simulink model "dcdc_buffer"  (R2026a)
settings: Solver=ode23tb  StopTime=simlength  FixedStep=tc  MaxStep=glb_time.tc
values from neighbouring files (symbols this model uses):
  afe_ctrl = ctrl_afe_setup(glb_time.ts_afe, grid_emu.omega_grid_nom)    [init_model_legacy.m]
  frequency_set = 300    [init_model_legacy.m]
  glb_time = timing_setup(fpwm_afe, trgo_afe, fpwm_inv, trgo_inv, fpwm_single_phase_inv, trgo_single_phase_inv, fpwm_dab, trgo_dab,      fpwm_psfbc, trgo_psfbc, fpwm_isop_rail, trgo_isop_rail, fpwm_cllc, trgo_cllc, t_measure, tc_factor, tc_decimation, delay_pwm, dead_time_afe,      dead_time_inv, dead_time_single_phase_inv, dead_time_dab, dead_time_psfbc, dead_time_isop_rail, dead_time_cllc)    [init_model_legacy.m]
  grid_emu = grid_three_phase_emulator('Dyn11', delta_star, grid_nominal_power, application_voltage, us1, us2, fgrid,                  eq_grid_inductance, eq_grid_resistance, eta, ucc, i1m, p_iron, n1, n2, core_area, core_length, mur,                  up_xi_pu_ref, up_eta_pu_ref, un_xi_pu_ref, un_eta_pu_ref)    [init_model_legacy.m]
  heatsink = liquid_cooled_plate_2kw_setup(weight, no_weight, cp_al, heat_capacity_hs, thermal_conductivity_al,      Rth_switch_HA, Rth_mosfet_HA, Rth_diode_HA, Tambient, DThs_init)    [init_model_legacy.m]
  Tambient = 40    [init_model_legacy.m]
undefined symbols (not defined in the file or in its folder): hwdata, igbt, magnitude
libraries: fl_lib x113, nesl_utility x63, igbt_simple_2th_lib x4, ee_lib x2, pi_ctrl x2, dq_vector_pi x1, linear_double_integrator_observer_ccaller x1, phase_shift_filter_ccaller x1, discrete_time_low_pass_filter x1, single_phase_pwm_modulator x1, three_phase_voltage_with_frt_emulator x1
(part 1 of 4)
settings Model: SimulationMode=accelerator  Creator=LTNBDA  LastModifiedBy=ltnbda
settings SolverCC: ZeroCrossControl=DisableAll  ZeroCrossAlgorithm=Adaptive  SolverResetMethod=Robust
settings DataIOCC: MaxDataPoints=1  SignalLoggingSaveFormat=ModelDataLogs
settings OptimizationCC: InitFltsAndDblsToZero=on  EfficientMapNaN2IntZero=off
settings DebuggingCC: SaveWithParameterizedLinksMsg=none  SignalResolutionControl=TryResolveAllWithWarning  IgnoredZcDiagnostic=none  MultiTaskDSMMsg=warning  MultiTaskCondExecSysMsg=none  MultiTaskRateTransMsg=warning
settings HardwareCC: ProdBitPerLong=64.0  ProdHWDeviceType=Generic->64-bit Embedded Processor (LP64)  TargetBitPerPointer=64.0  TargetBitPerSizeT=64.0  TargetBitPerPtrDiffT=64.0  TargetLongLongMode=on  TargetIntDivRoundTo=Zero  TargetEndianess=LittleEndian  TargetWordSize=64.0  TargetHWDeviceType=MATLAB Host  ProdEqTarget=off
settings SFSimCC: SimCustomHeaderCode=|
  | #include "phase_shift_flt_simulink.h"
  | #include "sv_pwm.h"
  | #include "rpi.h"
  | #include "rpi_simulink.h"
  | #include "first_harmonic_tracker.h"
  | #include "dqvector_pi.h"
  | #include "dqvector_pi_simulink.h"
  | #include "sv_pwm_simulink.h"
  | #include "dqpll_grid.h"
  | #include "first_harmonic_tracker_simulink.h"
  | #include "dqpll_grid_simulink.h"
  | #include "phase_shift_flt.h"
  | #include "math_f.h"
  | #include "linear_double_integrator_observer_simulink.h"
  | #include "linear_double_integrator_observer.h"
  | #include "sogi_flt_simulink.h"
  | #include "sogi_flt.h"
settings SFSimCC: SimUserSources=|
  | "rpi.c"
  | "rpi_simulink.c"
  | "dqvector_pi_simulink.c"
  | "dqvector_pi.c"
  | "sv_pwm_simulink.c"
  | "sv_pwm.c"
  | "first_harmonic_tracker_simulink.c"
  | "first_harmonic_tracker.c"
  | "dqpll_grid_simulink.c"
  | "dqpll_grid.c"
  | "phase_shift_flt_simulink.c"
  | "phase_shift_flt.c"
  | "linear_double_integrator_observer_simulink.c"
  | "linear_double_integrator_observer.c"
  | "sogi_flt_simulink.c"
  | "sogi_flt.c"
settings SFSimCC: SimUserIncludeDirs=|
  | include
  | src
settings CodeAppCC: MaxIdLength=128.0
settings GRTTargetCC: CombineOutputUpdateFcns=off  GRTInterface=on
settings SimscapeCC: SimscapeNormalizeSystem=off  SimscapeNominalValues="[{\"value\":\"1\",\"unit\":\"A\"},{\"value\":\"1\",\"unit\":\"bar\"},{\"value\":\"1\",\"unit\":\"cm^2\"},{\"value\":\"1\",\"unit\":\"cm^3/s\"},{\"value\":\"1\",\"unit\":\"kJ/kg\"},{\"value\":\"1\",\"unit\":\"kW\"},{\"value\":\"1\",\"unit\":\"l\"},{\"value\":\"1\",\"unit\":\"N\"},{\"value\":\"1\",\"unit\":\"N*m\"},{\"value\":\"1\",\"unit\":\"V\"}]"  SimscapeLogType=none  SimscapeLogDataHistory=5000.0

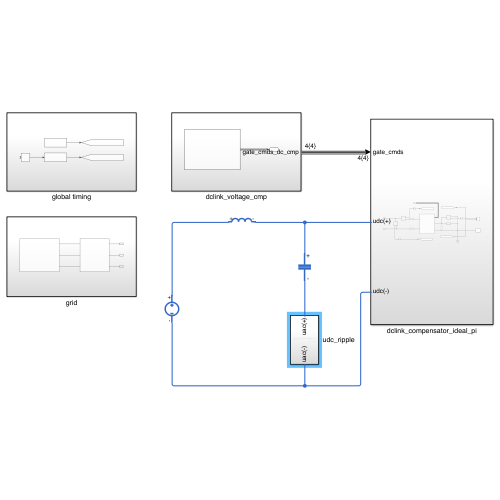
[thumbnail: Simulink's stored preview of the top-level diagram]
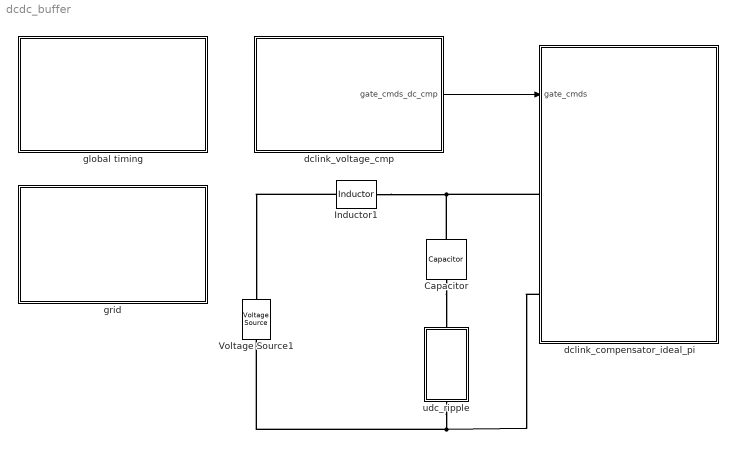
== system dcdc_buffer ==
  Capacitor : fl_lib/Electrical/Electrical Elements/Capacitor  c=7.2e-3 F  r=1e-6 Ohm  g=0 1/Ohm  i_specify=off  i_priority=None  i=0 A  i_nominal_specify=off  i_nominal_value=1  i_nominal_unit=A  v_specify=off  v_priority=None  v=0 V  v_nominal_specify=off  v_nominal_value=1  v_nominal_unit=V  vc_specify=off  vc_priority=High  vc=0 V  vc_nominal_specify=off  vc_nominal_value=1  vc_nominal_unit=V
  Inductor1 : fl_lib/Electrical/Electrical Elements/Inductor  l=250e-6 H  r=50e-3 Ohm  g=1e-9 1/Ohm  i_specify=off  i_priority=None  i=0 A  i_nominal_specify=off  i_nominal_value=1  i_nominal_unit=A  v_specify=off  v_priority=None  v=0 V  v_nominal_specify=off  v_nominal_value=1  v_nominal_unit=V  i_L_specify=off  i_L_priority=High  i_L=0 A  i_L_nominal_specify=off  i_L_nominal_value=1  i_L_nominal_unit=A
  Voltage Source1 : ee_lib/Sources/Voltage Source  dc_voltage=hwdata.single_phase_inverter.udc_nom V  ac_voltage=0 V  ac_shift=0 rad  ac_frequency=0 Hz  noise_mode=ee.enum.sources.noise.Disabled  PSD=0 V^2/Hz  sample_time=1e-3 s  repeatability=ee.enum.sources.repeatability.NotRepeatable  user_seed=0  auto_seed=3890346746  i_specify=off  i_priority=None  i=0 A  i_nominal_specify=off  i_nominal_value=1  i_nominal_unit=A  v_specify=off  v_priority=None  v=0 V  v_nominal_specify=off  v_nominal_value=1  v_nominal_unit=V
  dclink_compensator_ideal_pi : Subsystem
  dclink_voltage_cmp : Subsystem
  global timing : Subsystem
  grid : Subsystem
  udc_ripple : Subsystem
  wires:
  dclink_voltage_cmp/1(gate_cmds_dc_cmp) -> dclink_compensator_ideal_pi/1(gate_cmds)
  connections:
  dclink_compensator_ideal_pi/LConn1 -- Inductor1/RConn1 -- Capacitor/LConn1
  Inductor1/LConn1 -- Voltage Source1/LConn1
  Capacitor/RConn1 -- udc_ripple/LConn1
  udc_ripple/RConn1 -- Voltage Source1/RConn1 -- dclink_compensator_ideal_pi/LConn2

== system dcdc_buffer/dclink_compensator_ideal_pi ==
  gate_cmds : Inport
  Capacitor : fl_lib/Electrical/Electrical Elements/Capacitor  c=12e-3 F  r=1e-6 Ohm  g=0 1/Ohm  i_specify=off  i_priority=None  i=0 A  i_nominal_specify=off  i_nominal_value=1  i_nominal_unit=A  v_specify=off  v_priority=None  v=0 V  v_nominal_specify=off  v_nominal_value=1  v_nominal_unit=V  vc_specify=off  vc_priority=High  vc=0 V  vc_nominal_specify=off  vc_nominal_value=1  vc_nominal_unit=V
  Current Sensor : fl_lib/Electrical/Electrical Sensors/Current Sensor
  Electrical Reference1 : fl_lib/Electrical/Electrical Elements/Electrical Reference
  Inductor : fl_lib/Electrical/Electrical Elements/Inductor  l=250e-6 H  r=4e-3 Ohm  g=1e-9 1/Ohm  i_specify=off  i_priority=None  i=0 A  i_nominal_specify=off  i_nominal_value=1  i_nominal_unit=A  v_specify=off  v_priority=None  v=0 V  v_nominal_specify=off  v_nominal_value=1  v_nominal_unit=V  i_L_specify=off  i_L_priority=High  i_L=0 A  i_L_nominal_specify=off  i_L_nominal_value=1  i_L_nominal_unit=A
  Inductor1 : fl_lib/Electrical/Electrical Elements/Inductor  l=250e-6 H  r=4e-3 Ohm  g=1e-9 1/Ohm  i_specify=off  i_priority=None  i=0 A  i_nominal_specify=off  i_nominal_value=1  i_nominal_unit=A  v_specify=off  v_priority=None  v=0 V  v_nominal_specify=off  v_nominal_value=1  v_nominal_unit=V  i_L_specify=off  i_L_priority=High  i_L=0 A  i_L_nominal_specify=off  i_L_nominal_value=1  i_L_nominal_unit=A
  PS-Simulink Converter : nesl_utility/PS-Simulink Converter  PhysicalDomain=network_engine_domain  SubClassName=ps_output  LeftPortType=input  RightPortType=output  PseudoPeriodic=off  Frequencies=[]  VectorFormat=1-D array  Unit=A  AffineConversion=off
  PS-Simulink Converter1 : nesl_utility/PS-Simulink Converter  PhysicalDomain=network_engine_domain  SubClassName=ps_output  LeftPortType=input  RightPortType=output  PseudoPeriodic=off  Frequencies=[]  VectorFormat=1-D array  Unit=V  AffineConversion=off
  PS-Simulink Converter2 : nesl_utility/PS-Simulink Converter  PhysicalDomain=network_engine_domain  SubClassName=ps_output  LeftPortType=input  RightPortType=output  PseudoPeriodic=off  Frequencies=[]  VectorFormat=1-D array  Unit=V  AffineConversion=off
  Solver Configuration : nesl_utility/Solver Configuration  PhysicalDomain=network_engine_domain  SubClassName=solver  LeftPortType=input  RightPortType=generic  Tones=[]  Harmonics=[]  SimulateNoise=off  Profile=off  UseLocalSampling=off  EnableSwitchedLinearOptims=on  FrequencyDomain=off  UseCCode=off  RelTol=0.001  AbsTol=0.001  MinStep=1e-09  ToWorkspace=off  RevertToSquareIcSolve=off  NumHomotopyIterations=100  PhasorMode=off  PhasorModeNumHarmonics=1  ConsistencySolver=NEWTON_FTOL  CanonicalOrdering=UNORDERED  OptimizeIntermediates=UNOPTIMIZED  IndexReductionMethod=DerivativeReplacement  DoDC=off  ResidualTolerance=1e-4  ConsistencyTolSource=GLOBAL  ConsistencyAbsTol=0.001  ConsistencyRelTol=0.001  ConsistencyTolFactor=0.001  UseLocalSolver=on  LocalSolverChoice=NE_BACKWARD_EULER_ADVANCER  ResolveIndetEquations=on  FunctionEvalNumThread=1  LocalSolverSampleTime=glb_time.tc  DoFixedCost=on  MaxNonlinIter=nonlinear_iterations  MaxModeIter=2  ComputeImpulses=off  ImpulseIterations=2  LinearAlgebra=auto  LinearAlgebraNumThread=0  EquationFormulation=NE_TIME_EF  DelaysMemoryBudget=1024  AutomaticFiltering=on  FilteringTimeConstant=0.001  PartitionStorageMethod=AS_NEEDED  PartitionMemoryBudget=1024  PartitionMethod=ROBUST  MultibodyUseLocalSolver=off  MultibodyLocalSolverChoice=ODE1  MultibodyLocalSolverSampleTime=0.001
  Voltage Sensor : fl_lib/Electrical/Electrical Sensors/Voltage Sensor
  Voltage Sensor1 : fl_lib/Electrical/Electrical Sensors/Voltage Sensor
  Voltage Source : ee_lib/Sources/Voltage Source  Commented=on  dc_voltage=2000 V  ac_voltage=0 V  ac_shift=0 rad  ac_frequency=0 Hz  noise_mode=ee.enum.sources.noise.Disabled  PSD=0 V^2/Hz  sample_time=1e-3 s  repeatability=ee.enum.sources.repeatability.NotRepeatable  user_seed=0  auto_seed=3499211588  i_specify=off  i_priority=None  i=0 A  i_nominal_specify=off  i_nominal_value=1  i_nominal_unit=A  v_specify=off  v_priority=None  v=0 V  v_nominal_specify=off  v_nominal_value=1  v_nominal_unit=V
  single_phase_inverter : Subsystem
  udc_buffer : Scope  NumInputPorts=2
      settings: ActiveDisplayYMinimum=-428.225155436671  ActiveDisplayYMaximum=3854.02639893004  DataLoggingVariableName=ScopeData16
  udc(+) : PMIOPort  Side=Left
  udc(-) : PMIOPort  Port=2  Side=Left
  tag scope: dclink_voltage=global, i_buffer_glb=global, udc_buffer_glb=global
  wires:
  gate_cmds/1 -> single_phase_inverter/1(gate_cmds)
  PS-Simulink Converter/1 -> [i_buffer_glb]
  PS-Simulink Converter1/1 -> [udc_buffer_glb], udc_buffer/1  "udc_buffer_glb"
  [i_buffer_glb] -> udc_buffer/2  "i_buffer_glb"
  PS-Simulink Converter2/1 -> [dclink_voltage]  "dclink_voltage"
  connections:
  Inductor1/RConn1 -- Voltage Sensor1/RConn2 -- udc(-)/RConn1
  single_phase_inverter/RConn1 -- Inductor/RConn1
  single_phase_inverter/RConn2 -- Inductor1/LConn1
  Voltage Source/LConn1 -- Voltage Sensor/LConn1 -- Capacitor/LConn1 -- single_phase_inverter/LConn1
  Voltage Source/RConn1 -- Capacitor/RConn1 -- Voltage Sensor/RConn2 -- Electrical Reference1/LConn1 -- Solver Configuration/RConn1 -- single_phase_inverter/LConn2
  Current Sensor/RConn2 -- Inductor/LConn1
  udc(+)/RConn1 -- Voltage Sensor1/LConn1 -- Current Sensor/LConn1
  Current Sensor/RConn1 -- PS-Simulink Converter/LConn1
  PS-Simulink Converter1/LConn1 -- Voltage Sensor/RConn1
  PS-Simulink Converter2/LConn1 -- Voltage Sensor1/RConn1

== system dcdc_buffer/dclink_voltage_cmp ==
  dclink_cmp : Subsystem
  gate_cmds_dc_cmp : Outport
  wires:
  dclink_cmp/1(gate_cmds_dc_comp) -> gate_cmds_dc_cmp/1

== system dcdc_buffer/global timing ==
  Unit Delay : UnitDelay  SampleTime=glb_time.tc
  time_afe1 : Subsystem  mask{k=1}
      mask prompts: k "Time Gain"
      mask Display:
      | disp('time-gen');
      | port_label('input', 1, 'crt');
      | port_label('output', 1, 'tout');
  time_afe3 : Subsystem  mask{k=1}
      mask prompts: k "Time Gain"
      mask Display:
      | disp('time-gen');
      | port_label('output', 1, 'tout');
  tag scope: master_time=global, time_afe_module_1=global
  wires:
  time_afe1/1(Out1) -> [time_afe_module_1]
  time_afe3/1(Out1) -> [master_time]
  Unit Delay/1 -> time_afe1/1(correction_time)

== system dcdc_buffer/grid ==
  Open Circuit : fl_lib/Electrical/Electrical Elements/Open Circuit  v_specify=off  v_priority=None  v=0 V  v_nominal_specify=off  v_nominal_value=1  v_nominal_unit=V
  Open Circuit1 : fl_lib/Electrical/Electrical Elements/Open Circuit  v_specify=off  v_priority=None  v=0 V  v_nominal_specify=off  v_nominal_value=1  v_nominal_unit=V
  Open Circuit2 : fl_lib/Electrical/Electrical Elements/Open Circuit  v_specify=off  v_priority=None  v=0 V  v_nominal_specify=off  v_nominal_value=1  v_nominal_unit=V
  grid_emulator : Subsystem
  threephase_vi_measures : Subsystem
  connections:
  threephase_vi_measures/LConn3 -- grid_emulator/RConn3
  threephase_vi_measures/LConn1 -- grid_emulator/RConn1
  threephase_vi_measures/LConn2 -- grid_emulator/RConn2
  Open Circuit1/LConn1 -- threephase_vi_measures/RConn1
  Open Circuit2/LConn1 -- threephase_vi_measures/RConn2
  threephase_vi_measures/RConn3 -- Open Circuit/LConn1

== system dcdc_buffer/udc_ripple ==
  Constant : Constant  Value=-2*pi/3
  Controlled Voltage Source : fl_lib/Electrical/Electrical Sources/Controlled Voltage Source
  Gain : Gain  Gain=150
  Gain1 : Gain  Gain=2
  Simulink-PS Converter : nesl_utility/Simulink-PS Converter  PhysicalDomain=network_engine_domain  SubClassName=ps_input  LeftPortType=input  RightPortType=output  PseudoPeriodic=off  Frequencies=[]  NoiseDistribution=none  NoiseParameters=[]  Unit=V  AffineConversion=off  FilteringAndDerivatives=provide  SimscapeFilterOrder=1  InputFilterTimeConstant=0.001  UdotUserProvided=0
  Sin : Trigonometry
  Sum : Sum  Inputs=|++
  uac(+) : PMIOPort  Side=Left
  uac(-) : PMIOPort  Port=2  Side=Right
  wires:
  Sin/1 -> Gain/1
  Gain/1 -> Simulink-PS Converter/1
  [phase_grid_emulator] -> Sum/1
  Sum/1 -> Gain1/1
  Constant/1 -> Sum/2
  Gain1/1 -> Sin/1
  connections:
  Controlled Voltage Source/LConn1 -- uac(+)/RConn1
  Controlled Voltage Source/RConn2 -- uac(-)/RConn1
  Simulink-PS Converter/RConn1 -- Controlled Voltage Source/RConn1

== system dcdc_buffer/dclink_compensator_ideal_pi/single_phase_inverter ==
  gate_cmds : Inport
  single phase inverter : Subsystem
      settings: PortSchema="{\"entries\":[{\"content\":{\"sides\":[{\"content\":{\"connectorIds\":[\"LConn1\",\"LConn2\"]},\"type\":\"ConnectorPlacement.EquallySpacedRectSide\",\"uuid\":\"4fcf4fea-d38f-431b-8a91-be3ce9782faf\"},{\"content\":{\"connectorIds\":[\"RConn1\",\"RConn2\"],\"side\":\"RIGHT\"},\"type\":\"ConnectorPlacement.EquallySpacedRectSide\",\"uuid\":\"0aa56277-92e9-4e3b-84c7-43398254a4d8\"},{\"content\":{\"connectorIds\":[\"In1\"],\"side\":\"TOP\"},\"type\":\"ConnectorPlacement.EquallySpacedRectSide\",\"uuid\":\"5cd150dc-bcaf-4cd7-b2a8-3db203726730\"}]},\"type\":\"ConnectorPlacement.EquallySpacedConnector\",\"uuid\":\"bf8194c4-c327-4d40-bea4-f1e7617f80b4\"}],\"packageUris\":[\"http://schema.mathworks.com/mf0/Connector/R2020b\"],\"version\":\"1.0\"}"
  uac(+) : PMIOPort  Side=Right
  uac(-) : PMIOPort  Port=2  Side=Right
  udc(+) : PMIOPort  Port=3  Side=Left
  udc(-) : PMIOPort  Port=4  Side=Left
  wires:
  gate_cmds/1 -> single phase inverter/1(gate_cmds)
  connections:
  single phase inverter/RConn1 -- udc(+)/RConn1
  single phase inverter/LConn2 -- uac(-)/RConn1
  uac(+)/RConn1 -- single phase inverter/LConn1
  single phase inverter/RConn2 -- udc(-)/RConn1

== system dcdc_buffer/dclink_voltage_cmp/dclink_cmp ==
  acquisition_and_scaling_current_buffer : Subsystem
  acquisition_and_scaling_dc_voltage : Subsystem
  acquisition_and_scaling_dc_voltage_buffer : Subsystem
  acquisition_and_scaling_grid_voltage_ac : Subsystem
  dclink_compensation_ctrl : Subsystem
  phase_grid_hat : Scope  NumInputPorts=2
      settings: ActiveDisplayYMinimum=-4.986486486486486  ActiveDisplayYMaximum=5.4864864864864868
  pwm modulator_dclink_compensator : Subsystem
  gate_cmds_dc_comp : Outport
  wires:
  [TRGO_AFE_1] -> dclink_compensation_ctrl/Trigger
  [dclink_voltage] -> acquisition_and_scaling_dc_voltage/1(in)
  acquisition_and_scaling_dc_voltage/1(out) -> dclink_compensation_ctrl/1(dclink_voltage_pu)  "dclink_voltage_pu"
  [i_buffer_glb] -> acquisition_and_scaling_current_buffer/1(in)
  acquisition_and_scaling_current_buffer/1(out) -> dclink_compensation_ctrl/2(i_buffer_pu)
  pwm modulator_dclink_compensator/1(gate_cmds) -> gate_cmds_dc_comp/1
  dclink_compensation_ctrl/1(u_ctrl_buffer) -> pwm modulator_dclink_compensator/1(vout)
  [udc_buffer_glb] -> acquisition_and_scaling_dc_voltage_buffer/1(in)
  acquisition_and_scaling_dc_voltage_buffer/1(out) -> dclink_compensation_ctrl/3(udc_buffer_pu)
  [ug_abc] -> acquisition_and_scaling_grid_voltage_ac/1(in)
  acquisition_and_scaling_grid_voltage_ac/1(out) -> dclink_compensation_ctrl/4(ugrid_pu)  "ug_abc"
  dclink_compensation_ctrl/2(phase_grid_hat) -> phase_grid_hat/1  "phase_grid_hat"
  [phase_grid_emulator] -> phase_grid_hat/2

== system dcdc_buffer/global timing/time_afe1 ==
  correction_time : Inport
  Constant : Constant
  Gain : Gain  Gain=k
  Product : Product
  Sum : Sum  Inputs=|++
  time_1 : Clock
  Out1 : Outport
  wires:
  time_1/1 -> Gain/1
  Gain/1 -> Product/1
  Product/1 -> Out1/1
  correction_time/1 -> Sum/1
  Sum/1 -> Product/2
  Constant/1 -> Sum/2

== system dcdc_buffer/global timing/time_afe3 ==
  Gain : Gain  Gain=k
  time_1 : Clock
  Out1 : Outport
  wires:
  Gain/1 -> Out1/1
  time_1/1 -> Gain/1

== system dcdc_buffer/grid/grid_emulator ==
  Bus Selector : BusSelector  OutputSignals=ua_grid_emu,ub_grid_emu,uc_grid_emu
  Bus Selector1 : BusSelector  OutputSignals=gamma_grid_emulator,omega_grid_emulator
  Controlled Voltage Source : fl_lib/Electrical/Electrical Sources/Controlled Voltage Source
  Controlled Voltage Source1 : fl_lib/Electrical/Electrical Sources/Controlled Voltage Source
  Controlled Voltage Source2 : fl_lib/Electrical/Electrical Sources/Controlled Voltage Source
  Electrical Reference : fl_lib/Electrical/Electrical Elements/Electrical Reference
  Simulink-PS Converter : nesl_utility/Simulink-PS Converter  PhysicalDomain=network_engine_domain  SubClassName=ps_input  LeftPortType=input  RightPortType=output  PseudoPeriodic=off  Frequencies=[]  NoiseDistribution=none  NoiseParameters=[]  Unit=V  AffineConversion=on  FilteringAndDerivatives=provide  SimscapeFilterOrder=1  InputFilterTimeConstant=0.001  UdotUserProvided=0
  Simulink-PS Converter1 : nesl_utility/Simulink-PS Converter  PhysicalDomain=network_engine_domain  SubClassName=ps_input  LeftPortType=input  RightPortType=output  PseudoPeriodic=off  Frequencies=[]  NoiseDistribution=none  NoiseParameters=[]  Unit=V  AffineConversion=on  FilteringAndDerivatives=provide  SimscapeFilterOrder=1  InputFilterTimeConstant=0.001  UdotUserProvided=0
  Simulink-PS Converter2 : nesl_utility/Simulink-PS Converter  PhysicalDomain=network_engine_domain  SubClassName=ps_input  LeftPortType=input  RightPortType=output  PseudoPeriodic=off  Frequencies=[]  NoiseDistribution=none  NoiseParameters=[]  Unit=V  AffineConversion=on  FilteringAndDerivatives=provide  SimscapeFilterOrder=1  InputFilterTimeConstant=0.001  UdotUserProvided=0
  Solver Configuration : nesl_utility/Solver Configuration  PhysicalDomain=network_engine_domain  SubClassName=solver  LeftPortType=input  RightPortType=generic  Tones=[]  Harmonics=[]  SimulateNoise=off  Profile=off  UseLocalSampling=off  EnableSwitchedLinearOptims=on  FrequencyDomain=off  UseCCode=off  RelTol=0.001  AbsTol=0.001  MinStep=1e-09  ToWorkspace=off  RevertToSquareIcSolve=off  NumHomotopyIterations=100  PhasorMode=off  PhasorModeNumHarmonics=1  ConsistencySolver=NEWTON_FTOL  CanonicalOrdering=UNORDERED  OptimizeIntermediates=UNOPTIMIZED  IndexReductionMethod=DerivativeReplacement  DoDC=off  ResidualTolerance=1e-4  ConsistencyTolSource=GLOBAL  ConsistencyAbsTol=0.001  ConsistencyRelTol=0.001  ConsistencyTolFactor=0.001  UseLocalSolver=on  LocalSolverChoice=NE_BACKWARD_EULER_ADVANCER  ResolveIndetEquations=on  FunctionEvalNumThread=1  LocalSolverSampleTime=glb_time.tc  DoFixedCost=on  MaxNonlinIter=nonlinear_iterations  MaxModeIter=2  ComputeImpulses=off  ImpulseIterations=2  LinearAlgebra=auto  LinearAlgebraNumThread=0  EquationFormulation=NE_TIME_EF  DelaysMemoryBudget=1024  AutomaticFiltering=on  FilteringTimeConstant=0.001  PartitionStorageMethod=AS_NEEDED  PartitionMemoryBudget=1024  PartitionMethod=ROBUST  MultibodyUseLocalSolver=off  MultibodyLocalSolverChoice=ODE1  MultibodyLocalSolverSampleTime=0.001
  three_phase_voltage_source_with_frt_emulator : three_phase_voltage_with_frt_emulator/three_phase_voltage_source_with_frt_emulator  nominal_frequency_m=grid_emu.fgrid_nom  nominal_voltage_m=grid_emu.us_primary_nom  Vemu_ref_norm_m=grid_emu.Vemu_ref_norm  vp_xi_pu_m=grid_emu.up_xi_pu_ref  vp_eta_pu_m=grid_emu.up_eta_pu_ref  vn_xi_pu_m=grid_emu.un_xi_pu_ref  vn_eta_pu_m=grid_emu.un_eta_pu_ref  Am=filters.afe.SOF_50Hz.ss_c.A  Bm=filters.afe.SOF_50Hz.ss_c.B  Cm=filters.afe.SOF_50Hz.ss_c.C  enable_frt_1_m=frt_data.enable_frt_1  enable_frt_2_m=frt_data.enable_frt_2  start_time_LVRT_m=frt_data.start_time_LVRT  end_time_LVRT_m=frt_data.end_time_LVRT  deepPOSxi_m=frt_data.deepPOSxi  deepPOSeta_m=frt_data.deepPOSeta  deepNEGxi_m=frt_data.deepNEGxi  deepNEGeta_m=frt_data.deepNEGeta  Amplitude_U_m=frt_data.Amplitude_U  Amplitude_V_m=frt_data.Amplitude_V  Amplitude_W_m=frt_data.Amplitude_W  t_ramp_m=frt_data.t_ramp  Phase_shift_m=frt_data.Phase_shift
  threephase_vi_measures : Subsystem
  u1 : PMIOPort  Side=Right
  u2 : PMIOPort  Port=2  Side=Right
  u3 : PMIOPort  Port=3  Side=Right
  tag scope: phase_grid_emulator=global, pulsation_grid_emulator=global
  wires:
  Bus Selector1/2 -> [pulsation_grid_emulator]  "<omega_grid_emulator>"
  Bus Selector1/1 -> [phase_grid_emulator]  "<gamma_grid_emulator>"
  Bus Selector/2 -> Simulink-PS Converter1/1  "<ub_grid_emu>"
  Bus Selector/3 -> Simulink-PS Converter2/1  "<uc_grid_emu>"
  three_phase_voltage_source_with_frt_emulator/1 -> Bus Selector1/1, Bus Selector/1
  Bus Selector/1 -> Simulink-PS Converter/1  "<ua_grid_emu>"
  connections:
  Simulink-PS Converter/RConn1 -- Controlled Voltage Source/RConn1
  Simulink-PS Converter1/RConn1 -- Controlled Voltage Source1/RConn1
  Simulink-PS Converter2/RConn1 -- Controlled Voltage Source2/RConn1
  Controlled Voltage Source/RConn2 -- Controlled Voltage Source1/RConn2 -- Solver Configuration/RConn1 -- Electrical Reference/LConn1 -- Controlled Voltage Source2/RConn2
  u1/RConn1 -- threephase_vi_measures/RConn1
  u2/RConn1 -- threephase_vi_measures/RConn2
  u3/RConn1 -- threephase_vi_measures/RConn3
  Controlled Voltage Source/LConn1 -- threephase_vi_measures/LConn1
  Controlled Voltage Source1/LConn1 -- threephase_vi_measures/LConn2
  Controlled Voltage Source2/LConn1 -- threephase_vi_measures/LConn3

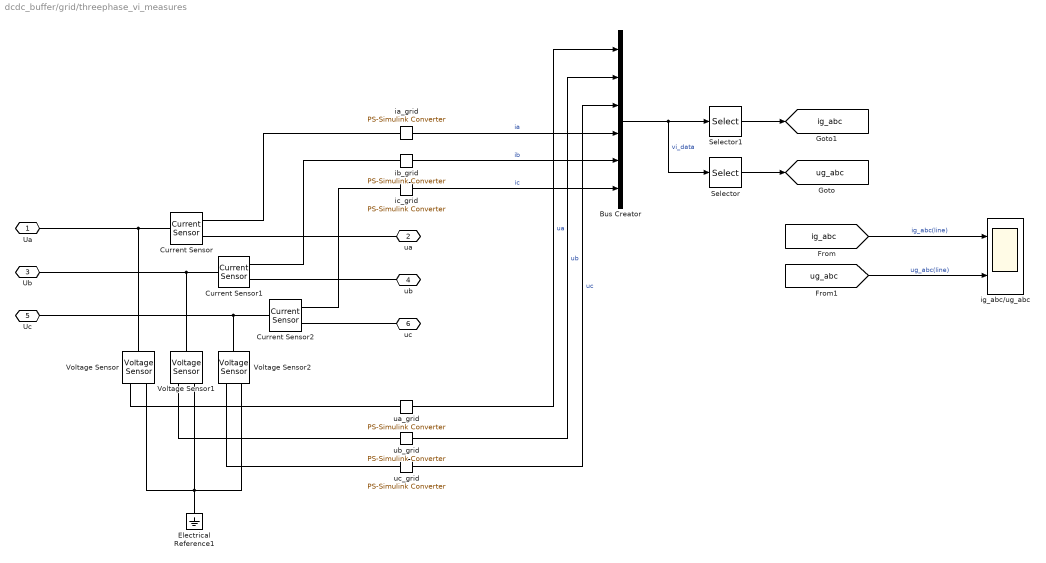
== system dcdc_buffer/grid/threephase_vi_measures ==
  Bus Creator : BusCreator  Inputs=6
  Current Sensor : fl_lib/Electrical/Electrical Sensors/Current Sensor
  Current Sensor1 : fl_lib/Electrical/Electrical Sensors/Current Sensor
  Current Sensor2 : fl_lib/Electrical/Electrical Sensors/Current Sensor
  Electrical Reference1 : fl_lib/Electrical/Electrical Elements/Electrical Reference
  Selector : Selector  InputPortWidth=6  IndexOptions=Index vector (dialog)  Indices=[1 2 3]  OutputSizes=1
  Selector1 : Selector  InputPortWidth=6  IndexOptions=Index vector (dialog)  Indices=[4 5 6]  OutputSizes=1
  Voltage Sensor : fl_lib/Electrical/Electrical Sensors/Voltage Sensor
  Voltage Sensor1 : fl_lib/Electrical/Electrical Sensors/Voltage Sensor
  Voltage Sensor2 : fl_lib/Electrical/Electrical Sensors/Voltage Sensor
  ia_grid : nesl_utility/PS-Simulink Converter  PhysicalDomain=network_engine_domain  SubClassName=ps_output  LeftPortType=input  RightPortType=output  PseudoPeriodic=off  Frequencies=[]  VectorFormat=1-D array  Unit=A  AffineConversion=off
  ib_grid : nesl_utility/PS-Simulink Converter  PhysicalDomain=network_engine_domain  SubClassName=ps_output  LeftPortType=input  RightPortType=output  PseudoPeriodic=off  Frequencies=[]  VectorFormat=1-D array  Unit=A  AffineConversion=off
  ic_grid : nesl_utility/PS-Simulink Converter  PhysicalDomain=network_engine_domain  SubClassName=ps_output  LeftPortType=input  RightPortType=output  PseudoPeriodic=off  Frequencies=[]  VectorFormat=1-D array  Unit=A  AffineConversion=off
  ig_abc/ug_abc : Scope  NumInputPorts=2
      settings: SampleTime=glb_time.tc  ActiveDisplayYMinimum=-662.618491750231  ActiveDisplayYMaximum=662.00821995187164  DataLoggingVariableName=ScopeData2
  ua_grid : nesl_utility/PS-Simulink Converter  PhysicalDomain=network_engine_domain  SubClassName=ps_output  LeftPortType=input  RightPortType=output  PseudoPeriodic=off  Frequencies=[]  VectorFormat=1-D array  Unit=V  AffineConversion=off
  ub_grid : nesl_utility/PS-Simulink Converter  PhysicalDomain=network_engine_domain  SubClassName=ps_output  LeftPortType=input  RightPortType=output  PseudoPeriodic=off  Frequencies=[]  VectorFormat=1-D array  Unit=V  AffineConversion=off
  uc_grid : nesl_utility/PS-Simulink Converter  PhysicalDomain=network_engine_domain  SubClassName=ps_output  LeftPortType=input  RightPortType=output  PseudoPeriodic=off  Frequencies=[]  VectorFormat=1-D array  Unit=V  AffineConversion=off
  Ua : PMIOPort  Side=Left
  ua : PMIOPort  Port=2  Side=Right
  Ub : PMIOPort  Port=3  Side=Left
  ub : PMIOPort  Port=4  Side=Right
  Uc : PMIOPort  Port=5  Side=Left
  uc : PMIOPort  Port=6  Side=Right
  tag scope: ig_abc=global, ug_abc=global
  wires:
  Bus Creator/1 -> Selector1/1, Selector/1  "vi_data"
  Selector/1 -> [ug_abc]
  ib_grid/1 -> Bus Creator/5  "ib"
  ia_grid/1 -> Bus Creator/4  "ia"
  ic_grid/1 -> Bus Creator/6  "ic"
  ua_grid/1 -> Bus Creator/1  "ua"
  ub_grid/1 -> Bus Creator/2  "ub"
  uc_grid/1 -> Bus Creator/3  "uc"
  Selector1/1 -> [ig_abc]
  [ug_abc] -> ig_abc/ug_abc/2  "ug_abc(line)"
  [ig_abc] -> ig_abc/ug_abc/1  "ig_abc(line)"
  connections:
  Current Sensor1/LConn1 -- Ub/RConn1 -- Voltage Sensor1/LConn1
  Electrical Reference1/LConn1 -- Voltage Sensor/RConn2 -- Voltage Sensor2/RConn2 -- Voltage Sensor1/RConn2
  Voltage Sensor/RConn1 -- ua_grid/LConn1
  Current Sensor/RConn2 -- ua/RConn1
  Voltage Sensor1/RConn1 -- ub_grid/LConn1
  Voltage Sensor2/LConn1 -- Current Sensor2/LConn1 -- Uc/RConn1
  Current Sensor/LConn1 -- Ua/RConn1 -- Voltage Sensor/LConn1
  Current Sensor1/RConn2 -- ub/RConn1
  Voltage Sensor2/RConn1 -- uc_grid/LConn1
  ib_grid/LConn1 -- Current Sensor1/RConn1
  ia_grid/LConn1 -- Current Sensor/RConn1
  ic_grid/LConn1 -- Current Sensor2/RConn1
  Current Sensor2/RConn2 -- uc/RConn1

== system dcdc_buffer/dclink_compensator_ideal_pi/single_phase_inverter/single phase inverter ==
  gate_cmds : Inport
  three_phase_inverter_with_igbt_simple_2th : Subsystem
  uac_out(+) : PMIOPort  Side=Left
  uac_out(-) : PMIOPort  Port=2  Side=Left
  udc(+) : PMIOPort  Port=3  Side=Right
  udc(-) : PMIOPort  Port=4  Side=Right
  wires:
  gate_cmds/1 -> three_phase_inverter_with_igbt_simple_2th/1(gate_cmds)
  connections:
  udc(-)/RConn1 -- three_phase_inverter_with_igbt_simple_2th/LConn2
  udc(+)/RConn1 -- three_phase_inverter_with_igbt_simple_2th/LConn1
  uac_out(+)/RConn1 -- three_phase_inverter_with_igbt_simple_2th/RConn1
  uac_out(-)/RConn1 -- three_phase_inverter_with_igbt_simple_2th/RConn2

== system dcdc_buffer/dclink_voltage_cmp/dclink_cmp/acquisition_and_scaling_current_buffer ==
  in : Inport
  1/Ti5 : Gain  Gain=1/750  SaturateOnIntegerOverflow=on  OutDataTypeStr=Inherit: Same as input  ParamDataTypeStr=Inherit: Same as input
  Quantizer : Quantizer  QuantizationInterval=adc12_quantization
  out : Outport
  wires:
  in/1 -> 1/Ti5/1
  1/Ti5/1 -> Quantizer/1
  Quantizer/1 -> out/1

== system dcdc_buffer/dclink_voltage_cmp/dclink_cmp/acquisition_and_scaling_dc_voltage ==
  in : Inport
  1/Ti3 : Gain  Gain=1/hwdata.single_phase_inverter.udc_nom  SaturateOnIntegerOverflow=on  OutDataTypeStr=Inherit: Same as input  ParamDataTypeStr=Inherit: Same as input
  Quantizer : Quantizer  QuantizationInterval=adc12_quantization
  out : Outport
  wires:
  in/1 -> 1/Ti3/1
  1/Ti3/1 -> Quantizer/1
  Quantizer/1 -> out/1

== system dcdc_buffer/dclink_voltage_cmp/dclink_cmp/acquisition_and_scaling_dc_voltage_buffer ==
  in : Inport
  1/Ti3 : Gain  Gain=1/hwdata.single_phase_inverter.udc_nom  SaturateOnIntegerOverflow=on  OutDataTypeStr=Inherit: Same as input  ParamDataTypeStr=Inherit: Same as input
  Quantizer : Quantizer  QuantizationInterval=adc12_quantization
  out : Outport
  wires:
  Quantizer/1 -> out/1
  1/Ti3/1 -> Quantizer/1
  in/1 -> 1/Ti3/1

== system dcdc_buffer/dclink_voltage_cmp/dclink_cmp/acquisition_and_scaling_grid_voltage_ac ==
  in : Inport
  1/Ti5 : Gain  Gain=1/grid_emu.u2bez  SaturateOnIntegerOverflow=on  OutDataTypeStr=Inherit: Same as input  ParamDataTypeStr=Inherit: Same as input
  Quantizer : Quantizer  QuantizationInterval=adc12_quantization
  out : Outport
  wires:
  Quantizer/1 -> out/1
  1/Ti5/1 -> Quantizer/1
  in/1 -> 1/Ti5/1

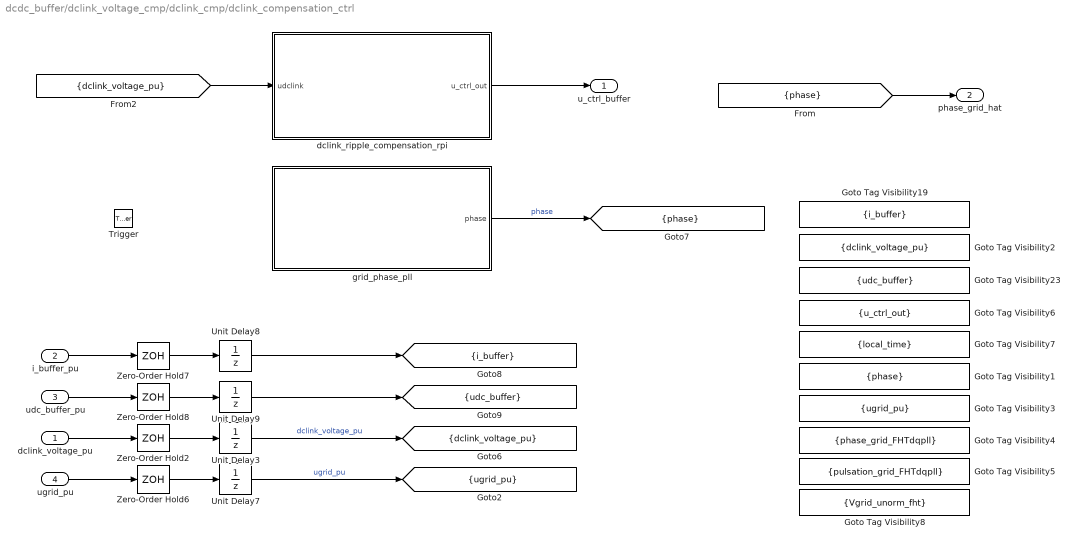
== system dcdc_buffer/dclink_voltage_cmp/dclink_cmp/dclink_compensation_ctrl ==
  dclink_voltage_pu : Inport
  i_buffer_pu : Inport  Port=2
  udc_buffer_pu : Inport  Port=3
  ugrid_pu : Inport  Port=4
  Trigger : TriggerPort  VariantControl=(inherit)  PortDimensions=1
  Goto Tag Visibility1 : GotoTagVisibility  GotoTag=phase
  Goto Tag Visibility19 : GotoTagVisibility  GotoTag=i_buffer
  Goto Tag Visibility2 : GotoTagVisibility  GotoTag=dclink_voltage_pu
  Goto Tag Visibility23 : GotoTagVisibility  GotoTag=udc_buffer
  Goto Tag Visibility3 : GotoTagVisibility  GotoTag=ugrid_pu
  Goto Tag Visibility4 : GotoTagVisibility  GotoTag=phase_grid_FHTdqpll
  Goto Tag Visibility5 : GotoTagVisibility  GotoTag=pulsation_grid_FHTdqpll
  Goto Tag Visibility6 : GotoTagVisibility  GotoTag=u_ctrl_out
  Goto Tag Visibility7 : GotoTagVisibility  GotoTag=local_time
  Goto Tag Visibility8 : GotoTagVisibility  GotoTag=Vgrid_unorm_fht
  Unit Delay{3,7..9} (4 alike) : UnitDelay  SampleTime=-1
  Zero-Order Hold{2,6..8} (4 alike) : ZeroOrderHold  SampleTime=-1
  dclink_ripple_compensation_rpi : Subsystem
  grid_phase_pll : Subsystem
  u_ctrl_buffer : Outport
  phase_grid_hat : Outport  Port=2
  tag scope: dclink_voltage_pu=scoped, i_buffer=scoped, phase=scoped, udc_buffer=scoped, ugrid_pu=scoped
  wires:
  dclink_voltage_pu/1 -> Zero-Order Hold2/1
  Unit Delay3/1 -> [dclink_voltage_pu]  "dclink_voltage_pu"
  Zero-Order Hold2/1 -> Unit Delay3/1
  [dclink_voltage_pu] -> dclink_ripple_compensation_rpi/1(udclink)
  dclink_ripple_compensation_rpi/1(u_ctrl_out) -> u_ctrl_buffer/1
  Zero-Order Hold7/1 -> Unit Delay8/1
  i_buffer_pu/1 -> Zero-Order Hold7/1
  Unit Delay8/1 -> [i_buffer]
  Unit Delay9/1 -> [udc_buffer]
  udc_buffer_pu/1 -> Zero-Order Hold8/1
  Zero-Order Hold8/1 -> Unit Delay9/1
  ugrid_pu/1 -> Zero-Order Hold6/1
  Zero-Order Hold6/1 -> Unit Delay7/1
  Unit Delay7/1 -> [ugrid_pu]  "ugrid_pu"
  grid_phase_pll/1(phase) -> [phase]  "phase"
  [phase] -> phase_grid_hat/1

== system dcdc_buffer/dclink_voltage_cmp/dclink_cmp/pwm modulator_dclink_compensator ==
  vout : Inport
  Constant : Constant  Value=0
  Single phase two level PWM generator with global TRGO : single_phase_pwm_modulator/Single phase two level PWM generator with global TRGO  f=glb_time.fPWM_INV  m_up=0.98  m_low=0.02  dead_time=glb_time.dead_time_INV  pos_cmd_gate=18  neg_cmd_gate=-3  polarity=-1  tc=glb_time.tc  double_sampling=glb_time.TRGO_INV_double_update
  gate_cmds : Outport
  tag scope: TRGO_AFE_1=global
  wires:
  [time_afe_module_1] -> Single phase two level PWM generator with global TRGO/1
  Single phase two level PWM generator with global TRGO/2 -> gate_cmds/1
  Constant/1 -> Single phase two level PWM generator with global TRGO/2
  vout/1 -> Single phase two level PWM generator with global TRGO/3
  Single phase two level PWM generator with global TRGO/1 -> [TRGO_AFE_1]

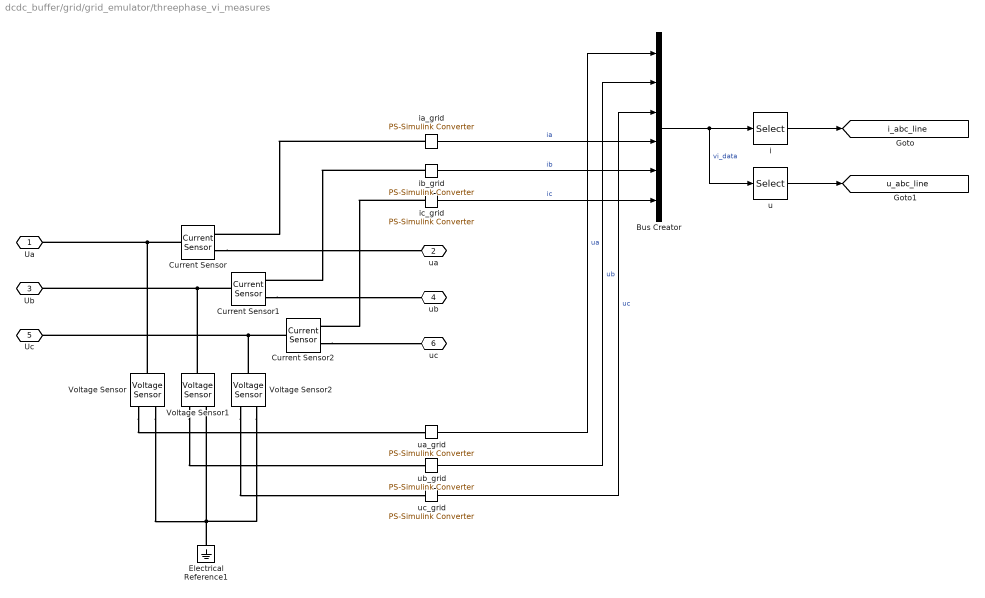
== system dcdc_buffer/grid/grid_emulator/threephase_vi_measures ==
  Bus Creator : BusCreator  Inputs=6
  Current Sensor : fl_lib/Electrical/Electrical Sensors/Current Sensor
  Current Sensor1 : fl_lib/Electrical/Electrical Sensors/Current Sensor
  Current Sensor2 : fl_lib/Electrical/Electrical Sensors/Current Sensor
  Electrical Reference1 : fl_lib/Electrical/Electrical Elements/Electrical Reference
  Voltage Sensor : fl_lib/Electrical/Electrical Sensors/Voltage Sensor
  Voltage Sensor1 : fl_lib/Electrical/Electrical Sensors/Voltage Sensor
  Voltage Sensor2 : fl_lib/Electrical/Electrical Sensors/Voltage Sensor
  i : Selector  InputPortWidth=6  IndexOptions=Index vector (dialog)  Indices=[4 5 6]  OutputSizes=1
  ia_grid : nesl_utility/PS-Simulink Converter  PhysicalDomain=network_engine_domain  SubClassName=ps_output  LeftPortType=input  RightPortType=output  PseudoPeriodic=off  Frequencies=[]  VectorFormat=1-D array  Unit=A  AffineConversion=off
  ib_grid : nesl_utility/PS-Simulink Converter  PhysicalDomain=network_engine_domain  SubClassName=ps_output  LeftPortType=input  RightPortType=output  PseudoPeriodic=off  Frequencies=[]  VectorFormat=1-D array  Unit=A  AffineConversion=off
  ic_grid : nesl_utility/PS-Simulink Converter  PhysicalDomain=network_engine_domain  SubClassName=ps_output  LeftPortType=input  RightPortType=output  PseudoPeriodic=off  Frequencies=[]  VectorFormat=1-D array  Unit=A  AffineConversion=off
  u : Selector  InputPortWidth=6  IndexOptions=Index vector (dialog)  Indices=[1 2 3]  OutputSizes=1
  ua_grid : nesl_utility/PS-Simulink Converter  PhysicalDomain=network_engine_domain  SubClassName=ps_output  LeftPortType=input  RightPortType=output  PseudoPeriodic=off  Frequencies=[]  VectorFormat=1-D array  Unit=V  AffineConversion=off
  ub_grid : nesl_utility/PS-Simulink Converter  PhysicalDomain=network_engine_domain  SubClassName=ps_output  LeftPortType=input  RightPortType=output  PseudoPeriodic=off  Frequencies=[]  VectorFormat=1-D array  Unit=V  AffineConversion=off
  uc_grid : nesl_utility/PS-Simulink Converter  PhysicalDomain=network_engine_domain  SubClassName=ps_output  LeftPortType=input  RightPortType=output  PseudoPeriodic=off  Frequencies=[]  VectorFormat=1-D array  Unit=V  AffineConversion=off
  Ua : PMIOPort  Side=Left
  ua : PMIOPort  Port=2  Side=Right
  Ub : PMIOPort  Port=3  Side=Left
  ub : PMIOPort  Port=4  Side=Right
  Uc : PMIOPort  Port=5  Side=Left
  uc : PMIOPort  Port=6  Side=Right
  tag scope: i_abc_line=global, u_abc_line=global
  wires:
  Bus Creator/1 -> i/1, u/1  "vi_data"
  ib_grid/1 -> Bus Creator/5  "ib"
  ia_grid/1 -> Bus Creator/4  "ia"
  ic_grid/1 -> Bus Creator/6  "ic"
  ua_grid/1 -> Bus Creator/1  "ua"
  ub_grid/1 -> Bus Creator/2  "ub"
  uc_grid/1 -> Bus Creator/3  "uc"
  i/1 -> [i_abc_line]
  u/1 -> [u_abc_line]
  connections:
  Current Sensor1/LConn1 -- Ub/RConn1 -- Voltage Sensor1/LConn1
  Electrical Reference1/LConn1 -- Voltage Sensor/RConn2 -- Voltage Sensor2/RConn2 -- Voltage Sensor1/RConn2
  Voltage Sensor/RConn1 -- ua_grid/LConn1
  Current Sensor/RConn2 -- ua/RConn1
  Voltage Sensor1/RConn1 -- ub_grid/LConn1
  Voltage Sensor2/LConn1 -- Current Sensor2/LConn1 -- Uc/RConn1
  Current Sensor/LConn1 -- Ua/RConn1 -- Voltage Sensor/LConn1
  Current Sensor1/RConn2 -- ub/RConn1
  Voltage Sensor2/RConn1 -- uc_grid/LConn1
  ib_grid/LConn1 -- Current Sensor1/RConn1
  ia_grid/LConn1 -- Current Sensor/RConn1
  ic_grid/LConn1 -- Current Sensor2/RConn1
  Current Sensor2/RConn2 -- uc/RConn1

== system dcdc_buffer/dclink_compensator_ideal_pi/single_phase_inverter/single phase inverter/three_phase_inverter_with_igbt_simple_2th ==
  gate_cmds : Inport
  full_bridge_with_igbt_simple_2th : Subsystem  mask{vce_sat_m=igbt.afe.Vce_sat, v_gamma_m=igbt.afe.Vdon_diode, Vth_gate_m=igbt.afe.Vth, Vth_gate_hyst_m=0.85, Eon_m=igbt.afe.Eon*1000, Eoff_m=igbt.afe.Eoff*1000, Err_m=igbt.afe.Erec*1000, Ic_ref_m=igbt.afe.Ion_sw_losses, Vdc_ref_m=igbt.afe.Voff_sw_losses, Vblock_Errf_m=50, rce_on_m=igbt.afe.Rce_on*1000, rd_on_m=igbt.afe.Rdon_diode*1000, Gce_off_m=1e-6, time_constant_edge_m=glb_time.tc, time_constant_ploss_m=1e3, Csnubber_m=igbt.afe.Csnubber_zvs, Rsnubber_m=igbt.afe.Rsnubber_zvs, rth_switch_JH_m=igbt.afe.Rth_switch_JH, rth_switch_HA_m=heatsink.Rth_switch_HA, rth_diode_JH_m=igbt.afe.Rth_diode_JH, rth_diode_HA_m=heatsink.Rth_diode_HA, JunctionTermalMass_m=igbt.afe.JunctionTermalMass, Tambient_m=Tambient, mass_heatsink_m=heatsink.no_weight, specific_heat_m=heatsink.cp}
      mask prompts: vce_sat_m "Collector-emitter on-stage voltage [V]"; v_gamma_m "Diode forward voltage [V]"; Vth_gate_m "Gate-emitter threshold voltage [V]"; Vth_gate_hyst_m "Half hysteresis band for the switching events [V]"; Eon_m "Turn-on energy at Ic_ref, Vdc_ref [mJ]"; Eoff_m "Turn-off energy at Ic_ref, Vdc_ref [mJ]"; Err_m "Reverse recovery energy at Ic_ref, Vdc_ref [mJ]"; Ic_ref_m "Reference current of the energies [A]"; Vdc_ref_m "Reference voltage of the energies [V]"; Vblock_Errf_m "V block Err"; rce_on_m "IGBT on-state series resistance [mOhm]"; rd_on_m "Diode series resistance [mOhm]"; Gce_off_m "Off-state conductance [1/Ohm]"; time_constant_edge_m "Sample&hold time constant (<< on-time) [us]"; time_constant_ploss_m "Loss averaging time constant (2-5 x Tsw) [us]"; Csnubber_m "Csnubber [F]"; Rsnubber_m "Rsnubber [Ohm]"; rth_switch_JH_m "Thermal impedance Junction-heatsink switch [K/W]"; rth_switch_HA_m "Thermal impedance heatsink-ambient switch[K/W]"; rth_diode_JH_m "Thermal impedance Junction-heatsink diode [K/W]"; rth_diode_HA_m "Thermal impedance heatsink-ambient diode [K/W]"; JunctionTermalMass_m "Junction Thermal Mass [J/K]"; Tambient_m "Ambient temperature [degC]"; mass_heatsink_m "Mass heatsink [kg]"; specific_heat_m "Specific heat capacity of the heatsink [J/K/Kg]"
  u1 : PMIOPort  Side=Right
  u2 : PMIOPort  Port=2  Side=Right
  udc(+) : PMIOPort  Port=3  Side=Left
  udc(-) : PMIOPort  Port=4  Side=Left
  wires:
  gate_cmds/1 -> full_bridge_with_igbt_simple_2th/1(gate_cmds)
  connections:
  u1/RConn1 -- full_bridge_with_igbt_simple_2th/RConn1
  u2/RConn1 -- full_bridge_with_igbt_simple_2th/RConn2
  udc(-)/RConn1 -- full_bridge_with_igbt_simple_2th/LConn2
  udc(+)/RConn1 -- full_bridge_with_igbt_simple_2th/LConn1

== system dcdc_buffer/dclink_voltage_cmp/dclink_cmp/dclink_compensation_ctrl/dclink_ripple_compensation_rpi ==
  udclink : Inport
  Sum : Sum  Inputs=++|
  alphabeta2dq : Subsystem
  dclink compensation : Scope  NumInputPorts=4
      settings: ActiveDisplayString=3  ActiveDisplayYMinimum=-0.32594771136796508  ActiveDisplayYMaximum=0.71408469991198853  DataLoggingVariableName=ScopeData11
  dclink compensation performance : Scope  NumInputPorts=4
      settings: ActiveDisplayString=3  ActiveDisplayYMinimum=-0.21051025390624994  ActiveDisplayYMaximum=1.89459228515625  DataLoggingVariableName=ScopeData10
  dq2alphabeta : Subsystem
  dq_vector_pi : Subsystem
  dx_dt : Subsystem
  idc_buffer_ctrl : Subsystem
  phase_shift_method_ccaller : Subsystem
  udc_buffer dclink voltage : Scope  NumInputPorts=3
      settings: ActiveDisplayYMinimum=-0.16107177734374997  ActiveDisplayYMaximum=1.44964599609375  DataLoggingVariableName=ScopeData9
  udc_buffer_ctrl : Subsystem
  u_ctrl_out : Outport
  wires:
  idc_buffer_ctrl/1(u_ctrl_out) -> u_ctrl_out/1, dclink compensation performance/4  "u_ctrl_out"
  dq_vector_pi/2(uq_ctrl) -> dclink compensation/4, dq2alphabeta/2(q)  "u:ctrl_buffer_q"
  dq_vector_pi/1(ud_ctrl) -> dclink compensation/3, dq2alphabeta/1(d)  "u:ctrl_buffer_d"
  alphabeta2dq/2("q ") -> dclink compensation/2, dq_vector_pi/2(q)  "i_buffer_q"
  alphabeta2dq/1("d ") -> dq_vector_pi/1(d), dclink compensation/1  "i_buffer_d"
  phase_shift_method_ccaller/2(y_out) -> alphabeta2dq/2(beta)
  phase_shift_method_ccaller/1(x_out) -> alphabeta2dq/1(alpha)
  udclink/1 -> dx_dt/1(x), dclink compensation performance/3, udc_buffer dclink voltage/2  "udc_dclink_pu"
  dx_dt/1(x_hat_ac) -> phase_shift_method_ccaller/1(x_in), dclink compensation performance/2  "udc_hat_pu"
  udc_buffer_ctrl/1(i_xi_ref) -> Sum/1  "i_buffer_ref"
  Sum/1 -> idc_buffer_ctrl/1(i_dc_buffer_ref), dclink compensation performance/1  "i_buffer_ref"
  [udc_buffer] -> udc_buffer_ctrl/1(udc_buffer_pu)
  [udc_buffer] -> udc_buffer dclink voltage/1  "udc_buffer_pu"
  dq2alphabeta/1(i_buffer_ref) -> Sum/2  "i_buffer_ref"
  [phase] -> udc_buffer dclink voltage/3  "phase_ripple"

== system dcdc_buffer/dclink_voltage_cmp/dclink_cmp/dclink_compensation_ctrl/grid_phase_pll ==
  FHT-PLL : Subsystem
  FHTdqpll : Scope  NumInputPorts=2
      settings: ActiveDisplayYMinimum=-1.624956414103508  ActiveDisplayYMaximum=4.624995157122612  DataLoggingVariableName=ScopeData3
  phase : Outport
  tag scope: phase_grid_FHTdqpll=scoped, pulsation_grid_FHTdqpll=scoped
  wires:
  FHT-PLL/1(phase_grid_fht_pll) -> [phase_grid_FHTdqpll]
  FHT-PLL/2(omega_grid_fht_pll) -> [pulsation_grid_FHTdqpll]
  [ugrid_pu] -> FHT-PLL/1(ug_abc_pu)
  [phase_grid_FHTdqpll] -> FHTdqpll/1  "phase_grid_FHTdqpll"
  [pulsation_grid_FHTdqpll] -> FHTdqpll/2  "pulsation_grid_FHTdqpll"
  [phase_grid_FHTdqpll] -> phase/1
